simulink model "sequence_detector1"  (R2025b)
settings: Solver=VariableStepAuto  StartTime=0.0  StopTime=10.0  RelTol=1e-3
libraries: simulink_extras x2
settings Model: Creator=hendl  LastModifiedBy=hendl

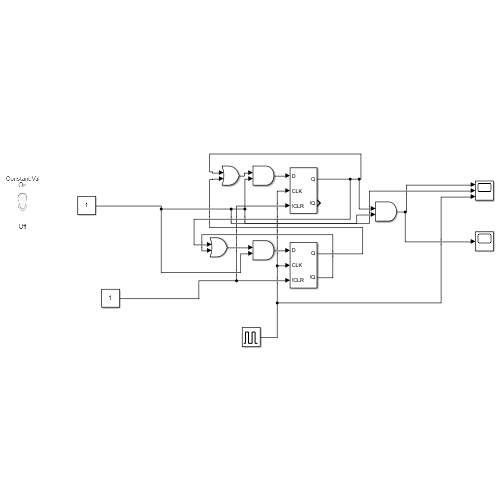
[thumbnail: Simulink's stored preview of the top-level diagram]
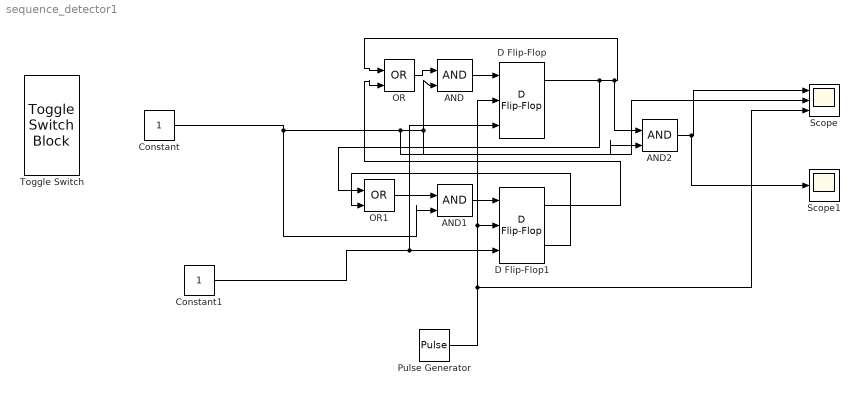
== system sequence_detector1 ==
  AND : Logic  IconShape=distinctive  AllPortsSameDT=off  OutDataTypeStr=boolean
  AND1 : Logic  IconShape=distinctive  AllPortsSameDT=off  OutDataTypeStr=boolean
  AND2 : Logic  IconShape=distinctive  AllPortsSameDT=off  OutDataTypeStr=boolean
  Constant : Constant  OutDataTypeStr=boolean
  Constant1 : Constant  OutDataTypeStr=boolean
  D Flip-Flop : simulink_extras/Flip Flops/D Flip-Flop
  D Flip-Flop1 : simulink_extras/Flip Flops/D Flip-Flop
  OR : Logic  Operator=OR  IconShape=distinctive  AllPortsSameDT=off  OutDataTypeStr=boolean
  OR1 : Logic  Operator=OR  IconShape=distinctive  AllPortsSameDT=off  OutDataTypeStr=boolean
  Pulse Generator : DiscretePulseGenerator  PulseType=Time based  Period=1  PulseWidth=50
  Scope : Scope  NumInputPorts=3
      settings: ActiveDisplayYMinimum=-0.12499999999999997  ActiveDisplayYMaximum=1.125
  Scope1 : Scope
      settings: ActiveDisplayYMinimum=-0.12499999999999997  ActiveDisplayYMaximum=1.125
  Toggle Switch : ToggleSwitchBlock
  wires:
  AND2/1 -> Scope1/1, Scope/1
  Constant/1 -> AND1/2, Scope/2, AND/2, AND2/2
  AND1/1 -> D Flip-Flop1/1
  Constant1/1 -> D Flip-Flop/3, D Flip-Flop1/3
  D Flip-Flop1/2 -> OR1/2
  Pulse Generator/1 -> Scope/3, D Flip-Flop/2, D Flip-Flop1/2
  D Flip-Flop/1 -> OR1/1, AND2/1, OR/1
  D Flip-Flop1/1 -> OR/2
  AND/1 -> D Flip-Flop/1
  OR/1 -> AND/1
  OR1/1 -> AND1/1
